simulink model "Robot1R_dyn"  (R2025b)
settings: Solver=VariableStepAuto  StartTime=0.0  StopTime=10.0  RelTol=1e-3  AbsTol=1e-3
undefined symbols (not defined in the file): X, Y, Z
libraries: sm_lib x13, nesl_utility x11, robotcorelib x1, simulink x1
settings Model: Creator=samu0  LastModifiedBy=samuisa
settings SolverCC: AutoScaleAbsTol=off  AlgebraicLoopSolver=TrustRegion  MaxZcPerStep=1.0
settings DebuggingCC: UnconnectedInputMsg=warning  UnconnectedOutputMsg=warning  UnconnectedLineMsg=warning  SymbolicDimsDataTypeCodeGenerationDiagnostic=none
settings ModelReferenceCC: EnableRefExpFcnMdlSchedulingChecks=on
settings SFSimCC: CustomCodeUndefinedFunction=UseInterfaceOnly
settings RTWCC: GPUComputeCapability=3.5  DLArmComputeVersion=19.05
settings SimscapeCC: SimscapeLogType=all  SimscapeLogSimulationStatistics=on  SimscapeLogDataHistory=10000.0

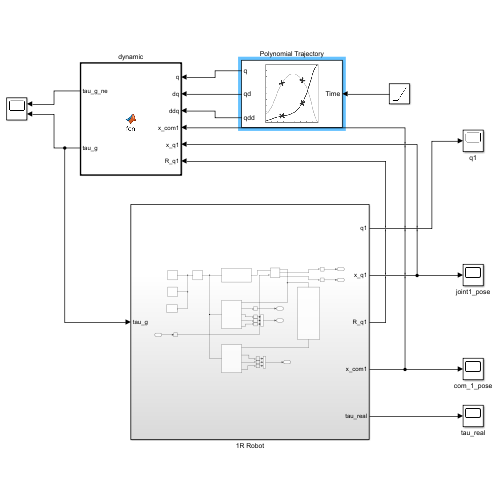
[thumbnail: Simulink's stored preview of the top-level diagram]
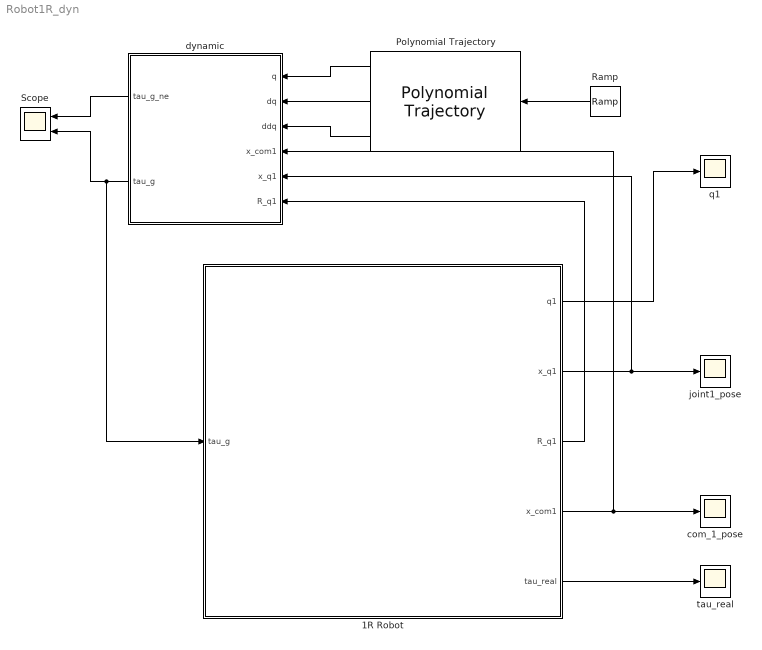
== system Robot1R_dyn ==
  1R Robot : Subsystem
  Polynomial Trajectory : robotcorelib/Polynomial Trajectory  WaypointSource=Internal  Waypoints=[ 0, 0.78 ]  TimePoints=[ 0, 10 ]  TimeInterval=[ 1, 4 ]  Method=Cubic Polynomial  ParameterSource=Internal  VelocityBoundaryCondition=zeros( 1,2 )  AccelerationBoundaryCondition=zeros( 2, 5 )  SimulateUsing=Interpreted execution
  Ramp : simulink/Sources/Ramp  slope=1  start=0  InitialOutput=0
  Scope : Scope  NumInputPorts=2
      settings: ActiveDisplayYMinimum=-12.780851676950455  ActiveDisplayYMaximum=52.28887020438399
  com_1_pose : Scope
      settings: DataLoggingVariableName=ScopeData4
  dynamic : MATLAB Function  TreatAsAtomicUnit=on
  joint1_pose : Scope
      settings: DataLoggingVariableName=ScopeData2
  q1 : Scope
  tau_real : Scope
      settings: DataLoggingVariableName=ScopeData3
  wires:
  1R Robot/1(q1) -> q1/1
  dynamic/1(tau_g_ne) -> Scope/1
  dynamic/2(tau_g) -> 1R Robot/1(tau_g), Scope/2
  1R Robot/3(R_q1) -> dynamic/6(R_q1)
  1R Robot/2(x_q1) -> dynamic/5(x_q1), joint1_pose/1
  1R Robot/4(x_com1) -> com_1_pose/1, dynamic/4(x_com1)
  1R Robot/5(tau_real) -> tau_real/1
  Polynomial Trajectory/3 -> dynamic/3(ddq)
  Polynomial Trajectory/2 -> dynamic/2(dq)
  Polynomial Trajectory/1 -> dynamic/1(q)
  Ramp/1 -> Polynomial Trajectory/1

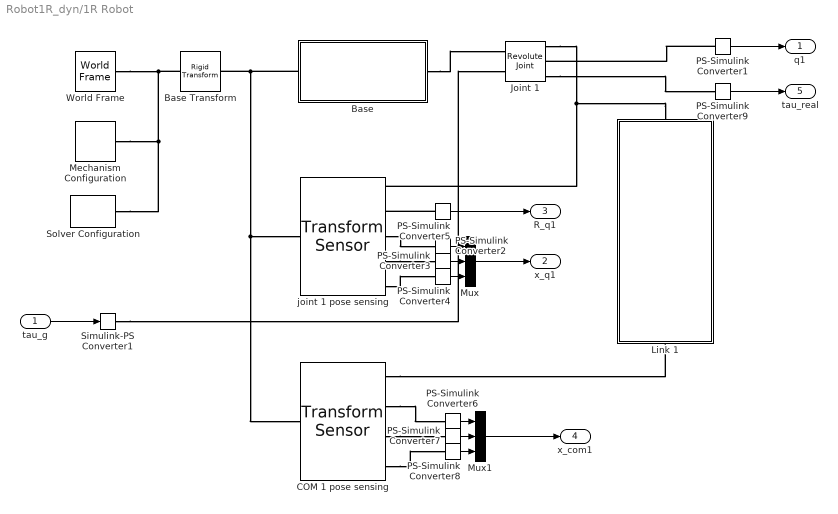
== system Robot1R_dyn/1R Robot ==
  tau_g : Inport
  Base : Subsystem
  Base Transform : sm_lib/Frames and Transforms/Rigid Transform  RotationMethod=AlignedAxes  FollAlignAxisA=+Z  BaseAlignAxisA=-Y  FollAlignAxisB=+X  BaseAlignAxisB=+X  RotationStandardAxis=+Z  RotationAngle=0  RotationAngleUnits=deg  RotationArbitraryAxis=[0 0 1]  RotationSequenceAxes=FollowerAxes  RotationSequence=XYX  RotationSequenceAngles=[0 0 0]  RotationSequenceAnglesUnits=deg  RotationMatrix=[1 0 0;0 1 0;0 0 1]  Quaternion=[1 0 0 0]  TranslationMethod=None  TranslationCartesianOffset=[0 0 0]  TranslationCartesianOffsetUnits=m  TranslationStandardAxis=+Z  TranslationStandardOffset=0  TranslationStandardOffsetUnits=m  TranslationROffset=0  TranslationROffsetUnits=m  TranslationThetaOffset=0  TranslationThetaOffsetUnits=deg  TranslationZOffset=0  TranslationZOffsetUnits=m
  COM 1 pose sensing : sm_lib/Frames and Transforms/Transform Sensor  MeasurementFrame=Base  RotationSequence=XYX  SenseAngle=off  SenseAxis=off  SenseQ=off  SenseR=off  SenseRotationSequence=off  SenseOmegaX=off  SenseOmegaY=off  SenseOmegaZ=off  SenseOmega=off  SenseQDot=off  SenseRDot=off  SenseRotationSequenceDot=off  SenseAlphaX=off  SenseAlphaY=off  SenseAlphaZ=off  SenseAlpha=off  SenseQDDot=off  SenseRDDot=off  SenseX=on  SenseY=on  SenseZ=on  SenseXYZ=off  SenseRad=off  SenseAzim=off  SenseDist=off  SenseInc=off  SenseXDot=off  SenseYDot=off  SenseZDot=off  SenseXYZDot=off  SenseRadDot=off  SenseAzimDot=off  SenseDistDot=off  SenseIncDot=off  SenseXDDot=off  SenseYDDot=off  SenseZDDot=off  SenseXYZDDot=off  SenseRadDDot=off  SenseAzimDDot=off  SenseDistDDot=off  SenseIncDDot=off
  Joint 1 : sm_lib/Joints/Revolute Joint  JointMode=Normal  CompositeWrenchDir=FollowerOnBase  CompositeWrenchFrame=BaseFrame  SenseConstraintForce=off  SenseConstraintTorque=off  SenseTotalForce=off  SenseTotalTorque=off  PositionTargetSpecify=on  PositionTargetPriority=High  PositionTargetValue=0  PositionTargetValueUnits=deg  VelocityTargetSpecify=off  VelocityTargetPriority=High  VelocityTargetValue=0  VelocityTargetValueUnits=deg/s  EquilibriumPosition=0  EquilibriumPositionUnits=rad  SpringStiffness=0  SpringStiffnessUnits=N*m/rad  DampingCoefficient=0.002  DampingCoefficientUnits=N*m*s/rad  LowerLimitSpecify=off  LowerLimitBound=-90  LowerLimitBoundUnits=deg  LowerLimitStiffness=1e4  LowerLimitStiffnessUnits=N*m/deg  LowerLimitDamping=10  LowerLimitDampingUnits=N*m/(deg/s)  LowerLimitTransitionRegionWidth=0.1  LowerLimitTransitionRegionWidthUnits=deg  UpperLimitSpecify=off  UpperLimitBound=90  UpperLimitBoundUnits=deg  UpperLimitStiffness=1e4  UpperLimitStiffnessUnits=N*m/deg  UpperLimitDamping=10  UpperLimitDampingUnits=N*m/(deg/s)  UpperLimitTransitionRegionWidth=0.1  UpperLimitTransitionRegionWidthUnits=deg  TorqueActuationMode=InputTorque  MotionActuationMode=ComputedMotion  SensePosition=on  SenseVelocity=off  SenseAcceleration=off  SenseTorqueForce=on  SenseLowerLimitTorqueForce=off  SenseUpperLimitTorqueForce=off
  Link 1 : Subsystem
  Mechanism Configuration : sm_lib/Utilities/Mechanism Configuration  UniformGravity=Constant  GravityVector=[0 0 -9.80665]  GravityVectorUnits=m/s^2  LinearizationDelta=0.001  JointModeTransitionNonlinearIterations=2
  Mux : Mux  Inputs=3
  Mux1 : Mux  Inputs=3
  PS-Simulink Converter{1..9} (9 alike) : nesl_utility/PS-Simulink Converter  PhysicalDomain=network_engine_domain  SubClassName=ps_output  LeftPortType=input  RightPortType=output  PseudoPeriodic=off  Frequencies=[]  VectorFormat=inherit  Unit=inherit  AffineConversion=off
  Simulink-PS Converter1 : nesl_utility/Simulink-PS Converter  PhysicalDomain=network_engine_domain  SubClassName=ps_input  LeftPortType=input  RightPortType=output  PseudoPeriodic=off  Frequencies=[]  NoiseDistribution=none  NoiseParameters=[]  Unit=1  AffineConversion=off  FilteringAndDerivatives=provide  SimscapeFilterOrder=1  InputFilterTimeConstant=0.001  UdotUserProvided=0
  Solver Configuration : nesl_utility/Solver Configuration  PhysicalDomain=network_engine_domain  SubClassName=solver  LeftPortType=input  RightPortType=generic  Tones=[]  Harmonics=[]  SimulateNoise=off  Profile=off  UseLocalSampling=off  EnableSwitchedLinearOptims=on  FrequencyDomain=off  UseCCode=off  RelTol=0.001  AbsTol=1e-06  MinStep=1e-09  ToWorkspace=off  RevertToSquareIcSolve=off  NumHomotopyIterations=100  PhasorMode=off  PhasorModeNumHarmonics=1  ConsistencySolver=NEWTON_XTOL_AFTER_FTOL  IndexReductionMethod=DerivativeReplacement  DoDC=off  ResidualTolerance=1e-09  ConsistencyTolSource=GLOBAL  ConsistencyAbsTol=0.001  ConsistencyRelTol=0.001  ConsistencyTolFactor=0.001  UseLocalSolver=off  LocalSolverChoice=NE_BACKWARD_EULER_ADVANCER  ResolveIndetEquations=on  FunctionEvalNumThread=1  LocalSolverSampleTime=0.001  DoFixedCost=off  MaxNonlinIter=3  MaxModeIter=2  ComputeImpulses=off  ImpulseIterations=2  LinearAlgebra=auto  LinearAlgebraNumThread=0  EquationFormulation=NE_TIME_EF  DelaysMemoryBudget=1024  AutomaticFiltering=on  FilteringTimeConstant=0.001  PartitionStorageMethod=AS_NEEDED  PartitionMemoryBudget=1024  PartitionMethod=ROBUST  MultibodyUseLocalSolver=off  MultibodyLocalSolverChoice=ODE1  MultibodyLocalSolverSampleTime=0.001
  World Frame : sm_lib/Frames and Transforms/World Frame
  joint 1 pose sensing : sm_lib/Frames and Transforms/Transform Sensor  MeasurementFrame=Base  RotationSequence=XYX  SenseAngle=off  SenseAxis=off  SenseQ=off  SenseR=on  SenseRotationSequence=off  SenseOmegaX=off  SenseOmegaY=off  SenseOmegaZ=off  SenseOmega=off  SenseQDot=off  SenseRDot=off  SenseRotationSequenceDot=off  SenseAlphaX=off  SenseAlphaY=off  SenseAlphaZ=off  SenseAlpha=off  SenseQDDot=off  SenseRDDot=off  SenseX=on  SenseY=on  SenseZ=on  SenseXYZ=off  SenseRad=off  SenseAzim=off  SenseDist=off  SenseInc=off  SenseXDot=off  SenseYDot=off  SenseZDot=off  SenseXYZDot=off  SenseRadDot=off  SenseAzimDot=off  SenseDistDot=off  SenseIncDot=off  SenseXDDot=off  SenseYDDot=off  SenseZDDot=off  SenseXYZDDot=off  SenseRadDDot=off  SenseAzimDDot=off  SenseDistDDot=off  SenseIncDDot=off
  q1 : Outport
  x_q1 : Outport  Port=2
  R_q1 : Outport  Port=3
  x_com1 : Outport  Port=4
  tau_real : Outport  Port=5
  wires:
  PS-Simulink Converter2/1 -> Mux/1
  PS-Simulink Converter7/1 -> Mux1/2
  tau_g/1 -> Simulink-PS Converter1/1
  Mux/1 -> x_q1/1
  PS-Simulink Converter4/1 -> Mux/3
  PS-Simulink Converter5/1 -> R_q1/1
  PS-Simulink Converter8/1 -> Mux1/3
  PS-Simulink Converter6/1 -> Mux1/1
  Mux1/1 -> x_com1/1
  PS-Simulink Converter1/1 -> q1/1
  PS-Simulink Converter3/1 -> Mux/2
  PS-Simulink Converter9/1 -> tau_real/1
  connections:
  Mechanism Configuration/RConn1 -- Base Transform/LConn1 -- World Frame/RConn1 -- Solver Configuration/RConn1
  Base Transform/RConn1 -- Base/LConn1 -- COM 1 pose sensing/LConn1 -- joint 1 pose sensing/LConn1
  Link 1/LConn1 -- Joint 1/RConn1 -- joint 1 pose sensing/RConn1
  PS-Simulink Converter1/LConn1 -- Joint 1/RConn2
  joint 1 pose sensing/RConn5 -- PS-Simulink Converter4/LConn1
  PS-Simulink Converter5/LConn1 -- joint 1 pose sensing/RConn2
  Simulink-PS Converter1/RConn1 -- Joint 1/LConn2
  COM 1 pose sensing/RConn2 -- PS-Simulink Converter6/LConn1
  COM 1 pose sensing/RConn4 -- PS-Simulink Converter8/LConn1
  COM 1 pose sensing/RConn3 -- PS-Simulink Converter7/LConn1
  joint 1 pose sensing/RConn3 -- PS-Simulink Converter2/LConn1
  Base/RConn1 -- Joint 1/LConn1
  joint 1 pose sensing/RConn4 -- PS-Simulink Converter3/LConn1
  COM 1 pose sensing/RConn1 -- Link 1/RConn1
  Joint 1/RConn3 -- PS-Simulink Converter9/LConn1

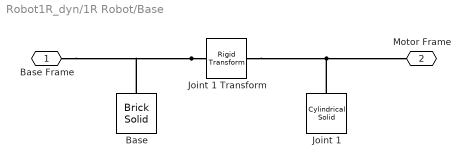
== system Robot1R_dyn/1R Robot/Base ==
  Base : sm_lib/Body Elements/Brick Solid  BrickDimensions=[5 5 0.5]  BrickDimensionsUnits=m  ExportEntireGeometry=off  InertiaType=PointMass  BasedOnType=Density  Density=1000  DensityUnits=kg/m^3  Mass=0  MassUnits=kg  CenterOfMass=[0 0 0]  CenterOfMassUnits=m  MomentsOfInertia=[1 1 1]  MomentsOfInertiaUnits=kg*m^2  ProductsOfInertia=[0 0 0]  ProductsOfInertiaUnits=kg*m^2  GraphicType=FromGeometry  MarkerShape=Sphere  MarkerSize=10  GraphicVisPropType=SimpleVisualProperties  GraphicDiffuseColor=[1 1 0]  GraphicOpacity=1  GraphicSpecularColor=[0.5 0.5 0.5 1.0]  GraphicAmbientColor=[0.15 0.15 0.15 1.0]  GraphicEmissiveColor=[0.0 0.0 0.0 1.0]  GraphicShininess=75  DoExposeReferenceFrame=on  SerializedFrames=<Frames/>
  Joint 1 : sm_lib/Body Elements/Cylindrical Solid  CylinderRadius=0.5  CylinderRadiusUnits=m  CylinderLength=0.6  CylinderLengthUnits=m  ExportEntireGeometry=off  InertiaType=PointMass  BasedOnType=Mass  Density=1000  DensityUnits=kg/m^3  Mass=0  MassUnits=kg  CenterOfMass=[0 0 0]  CenterOfMassUnits=m  MomentsOfInertia=[1 1 1]  MomentsOfInertiaUnits=kg*m^2  ProductsOfInertia=[0 0 0]  ProductsOfInertiaUnits=kg*m^2  GraphicType=FromGeometry  MarkerShape=Sphere  MarkerSize=10  GraphicVisPropType=SimpleVisualProperties  GraphicDiffuseColor=[1 0 1]  GraphicOpacity=1  GraphicSpecularColor=[0.5 0.5 0.5 1.0]  GraphicAmbientColor=[0.15 0.15 0.15 1.0]  GraphicEmissiveColor=[0.0 0.0 0.0 1.0]  GraphicShininess=75  DoExposeReferenceFrame=on  SerializedFrames=<Frames/>
  Joint 1 Transform : sm_lib/Frames and Transforms/Rigid Transform  RotationMethod=None  FollAlignAxisA=-Y  BaseAlignAxisA=+Y  FollAlignAxisB=+X  BaseAlignAxisB=+X  RotationStandardAxis=+Z  RotationAngle=0  RotationAngleUnits=deg  RotationArbitraryAxis=[0 0 1]  RotationSequenceAxes=FollowerAxes  RotationSequence=XYX  RotationSequenceAngles=[0 0 0]  RotationSequenceAnglesUnits=deg  RotationMatrix=[1 0 0;0 1 0;0 0 1]  Quaternion=[1 0 0 0]  TranslationMethod=StandardAxis  TranslationCartesianOffset=[0 0 0]  TranslationCartesianOffsetUnits=m  TranslationStandardAxis=+Z  TranslationStandardOffset=0.5  TranslationStandardOffsetUnits=m  TranslationROffset=0  TranslationROffsetUnits=m  TranslationThetaOffset=0  TranslationThetaOffsetUnits=deg  TranslationZOffset=0  TranslationZOffsetUnits=m
  Base Frame : PMIOPort  Side=Left
  Motor Frame : PMIOPort  Port=2  Side=Right
  connections:
  Joint 1 Transform/LConn1 -- Base Frame/RConn1 -- Base/RConn1
  Joint 1 Transform/RConn1 -- Motor Frame/RConn1 -- Joint 1/RConn1

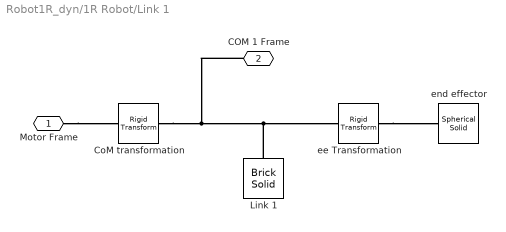
== system Robot1R_dyn/1R Robot/Link 1 ==
  CoM transformation : sm_lib/Frames and Transforms/Rigid Transform  RotationMethod=None  FollAlignAxisA=+X  BaseAlignAxisA=+Y  FollAlignAxisB=+Y  BaseAlignAxisB=+Z  RotationStandardAxis=+Z  RotationAngle=0  RotationAngleUnits=deg  RotationArbitraryAxis=[0 0 1]  RotationSequenceAxes=FollowerAxes  RotationSequence=XYX  RotationSequenceAngles=[0 0 0]  RotationSequenceAnglesUnits=deg  RotationMatrix=[1 0 0;0 1 0;0 0 1]  Quaternion=[1 0 0 0]  TranslationMethod=StandardAxis  TranslationCartesianOffset=[0 0 0]  TranslationCartesianOffsetUnits=m  TranslationStandardAxis=+X  TranslationStandardOffset=2.5  TranslationStandardOffsetUnits=m  TranslationROffset=0  TranslationROffsetUnits=m  TranslationThetaOffset=0  TranslationThetaOffsetUnits=deg  TranslationZOffset=0  TranslationZOffsetUnits=m
  Link 1 : sm_lib/Body Elements/Brick Solid  BrickDimensions=[5 0.5 0.5]  BrickDimensionsUnits=m  ExportEntireGeometry=off  InertiaType=CalculateFromGeometry  BasedOnType=Mass  Density=1000  DensityUnits=kg/m^3  Mass=1  MassUnits=kg  CenterOfMass=[0 0 0]  CenterOfMassUnits=m  MomentsOfInertia=[1 1 1]  MomentsOfInertiaUnits=kg*m^2  ProductsOfInertia=[0 0 0]  ProductsOfInertiaUnits=kg*m^2  GraphicType=FromGeometry  MarkerShape=Sphere  MarkerSize=10  GraphicVisPropType=SimpleVisualProperties  GraphicDiffuseColor=[1 0 0]  GraphicOpacity=1  GraphicSpecularColor=[0.5 0.5 0.5 1.0]  GraphicAmbientColor=[0.15 0.15 0.15 1.0]  GraphicEmissiveColor=[0.0 0.0 0.0 1.0]  GraphicShininess=75  DoExposeReferenceFrame=on  SerializedFrames=<Frames/>
  ee Transformation : sm_lib/Frames and Transforms/Rigid Transform  RotationMethod=None  FollAlignAxisA=+X  BaseAlignAxisA=+Y  FollAlignAxisB=+Y  BaseAlignAxisB=+Z  RotationStandardAxis=+Z  RotationAngle=0  RotationAngleUnits=deg  RotationArbitraryAxis=[0 0 1]  RotationSequenceAxes=FollowerAxes  RotationSequence=XYX  RotationSequenceAngles=[0 0 0]  RotationSequenceAnglesUnits=deg  RotationMatrix=[1 0 0;0 1 0;0 0 1]  Quaternion=[1 0 0 0]  TranslationMethod=StandardAxis  TranslationCartesianOffset=[0 0 0]  TranslationCartesianOffsetUnits=m  TranslationStandardAxis=+X  TranslationStandardOffset=2.5  TranslationStandardOffsetUnits=m  TranslationROffset=0  TranslationROffsetUnits=m  TranslationThetaOffset=0  TranslationThetaOffsetUnits=deg  TranslationZOffset=0  TranslationZOffsetUnits=m
  end effector : sm_lib/Body Elements/Spherical Solid  SphereRadius=0.5  SphereRadiusUnits=m  ExportEntireGeometry=off  InertiaType=PointMass  BasedOnType=Mass  Density=1000  DensityUnits=kg/m^3  Mass=0  MassUnits=kg  CenterOfMass=[0 0 0]  CenterOfMassUnits=m  MomentsOfInertia=[1 1 1]  MomentsOfInertiaUnits=kg*m^2  ProductsOfInertia=[0 0 0]  ProductsOfInertiaUnits=kg*m^2  GraphicType=FromGeometry  MarkerShape=Sphere  MarkerSize=10  GraphicVisPropType=SimpleVisualProperties  GraphicDiffuseColor=[0 0 1]  GraphicOpacity=1  GraphicSpecularColor=[0.5 0.5 0.5 1.0]  GraphicAmbientColor=[0.15 0.15 0.15 1.0]  GraphicEmissiveColor=[0.0 0.0 0.0 1.0]  GraphicShininess=75  DoExposeReferenceFrame=on  SerializedFrames=<Frames/>
  Motor Frame : PMIOPort  Side=Left
  COM 1 Frame : PMIOPort  Port=2  Side=Right
  connections:
  ee Transformation/RConn1 -- end effector/RConn1
  CoM transformation/RConn1 -- COM 1 Frame/RConn1 -- Link 1/RConn1 -- ee Transformation/LConn1
  Motor Frame/RConn1 -- CoM transformation/LConn1

== matlab function Robot1R_dyn/dynamic ==
  data: q input; dq input; tau_g_ne output; tau_g output; ddq input; x_com1 input; x_q1 input; R_q1 input
function [tau_g_ne, tau_g] = fcn(q, dq, ddq, x_com1, x_q1, R_q1)
    %%
    % ========================================================
    % INITIALIZATION
    % ========================================================
    m1 = 1;
    g_mag = 9.80665; % Magnitudo scalare per tau_g
    
    % Gravità modellata come accelerazione fittizia della base (VERSO L'ALTO)
    vdot_0 = [0; g_mag; 0]; 

    % Position vector of the COM with respect to joint 1 frame
    l1 = 2.5; 
    Pc1 = R_q1' * (x_com1 - x_q1);
    
    % Inertia tensor with respect to the COM
    ix = 0;
    iy = (1/12)*m1*(2*l1)^2;
    iz = (1/12)*m1*(2*l1)^2;
    I1 = [ix, 0, 0;
          0, iy, 0;
          0, 0, iz];
          
    % Z-axis vector for revolute joints (IN LOCAL FRAME!)
    Z1 = [0; 0; 1];
    
    % Kinematic conditions of the base (Link 0 assumed fixed)
    w_0 = [0; 0; 0];
    wdot_0 = [0; 0; 0];
    
    % Joint position vectors 
    P1 = [0; 0; 0.5];         % Posizione giunto 1 in frame 0 (se x_q1 è assoluto, usa x_q1)
    P2 = [2*l1; 0; 0];        % Joint 2 (end-effector) position with respect to frame 1
    
    % Forces and torques at the end-effector (f2, n2 assumed zero)
    f_2 = [0; 0; 0];
    n_2 = [0; 0; 0];
    % -------------------------------------------------------
            
    % R12: Rotation from frame 1 to frame 2 (assumed identity)
    R12 = eye(3); 
    
    %%
    % ========================================================
    % FORWARD RECURSIVE STEPS (From base to end-effector)
    % ========================================================
    
    % --- STEP 1: Angular velocity ---
    w_1 = R_q1' * w_0 + dq * Z1;
            
    % --- STEP 2: Angular acceleration ---
    wdot_1 = R_q1' * wdot_0 + cross(R_q1' * w_0, dq * Z1) + ddq * Z1;
               
    % --- STEP 3: Linear acceleration (Joint) ---
    % Usa P1 (o x_q1 se questo è il vettore corretto rispetto a frame 0)
    vdot_1 = R_q1' * (cross(wdot_0, P1) + cross(w_0, cross(w_0, P1)) + vdot_0);
                
    % --- STEP 4: Linear acceleration of the COM ---
    vdot_c1 = cross(wdot_1, Pc1) + cross(w_1, cross(w_1, Pc1)) + vdot_1;
                
    % --- STEP 5: Force acting on the COM ---
    F_1 = m1 * vdot_c1;
             
    % --- STEP 6: Torque acting about the COM ---
    N_1 = I1 * wdot_1 + cross(w_1, I1 * w_1);
    
    %%
    % ========================================================
    % BACKWARD RECURSIVE STEPS (From end-effector to base)
    % ========================================================
            
    % --- STEP 7: Force acting on the joint ---
    f_1 = R12 * f_2 + F_1;
    
    % --- STEP 8: Torque acting on the joint ---
    n_1 = N_1 + R12 * n_2 + cross(Pc1, F_1) + cross(P2, R12 * f_2);
            
    % --- STEP 9: Torque on the axis of motion (Z) ---
    tau_g_ne = n_1' * Z1; % Ora Z1 è [0;0;1], quindi estrae n_1(3)
    
    % --- SECONDARY OUTPUT ---
    % Gravity compensation torque solo statica (SCALARE!)
    tau_g = m1 * l1 * g_mag * cos(q);
    
end
